simulink library "sm_car_scene_crg_germania_f"  (R2026a)
settings: Solver=VariableStepAuto
undefined symbols (not defined in the file or in its folder): Scene
libraries: Scene_Utilities x3
Description:
  | Scene of Simscape Vehicle Templates Library
  | 
  | Copyright 2018-2024 The MathWorks, Inc.
settings Model: Creator=smiller  LastModifiedBy=andrei

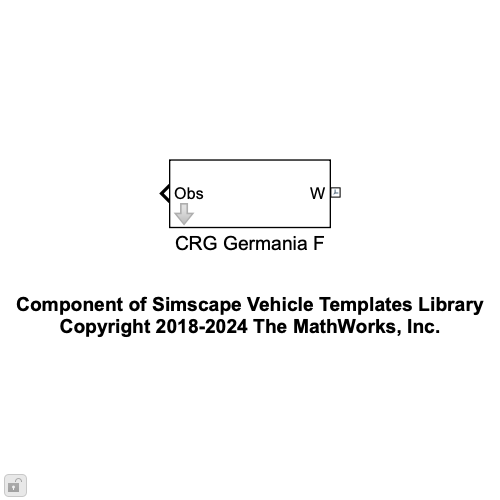
[thumbnail: Simulink's stored preview of the top-level diagram]
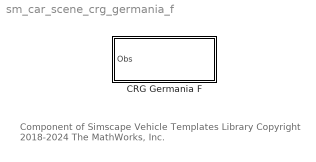
== system sm_car_scene_crg_germania_f ==
  note: Component of Simscape Vehicle Templates Library
      | Copyright 2018-2024 The MathWorks, Inc.
  CRG Germania F : Subsystem  mask{geometry=Scene.CRG_Germania_F.Geometry}
      mask prompts: geometry "Geometry (structure)"

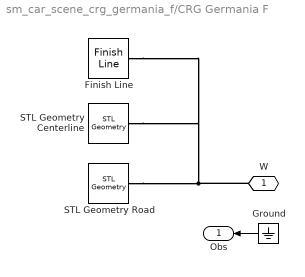
== system sm_car_scene_crg_germania_f/CRG Germania F ==
  Finish Line : Scene_Utilities/Finish Line  post_h=geometry.finish_line.post.height  post_r=geometry.finish_line.post.radius  line_w=geometry.finish_line.post.separation  post_clr=geometry.finish_line.post.clr  post_opc=geometry.finish_line.post.opc  offset_xyz=geometry.finish_line.offset.xyz  offset_yaw=geometry.finish_line.offset.yaw  offset_pitch=geometry.finish_line.offset.pitch  offset_roll=geometry.finish_line.offset.roll
  Ground : Ground
  STL Geometry Centerline : Scene_Utilities/STL Geometry  stl_file=geometry.centerline.filename  stl_units=geometry.centerline.fileunits  stl_clr=geometry.centerline.clr  stl_opc=geometry.centerline.opc  stl_x=geometry.centerline.x  stl_y=geometry.centerline.y  stl_z=geometry.centerline.z  stl_yaw=geometry.centerline.yaw  stl_pitch=geometry.centerline.pitch  stl_roll=geometry.centerline.roll
  STL Geometry Road : Scene_Utilities/STL Geometry  stl_file=geometry.filename  stl_units=geometry.fileunits  stl_clr=geometry.clr  stl_opc=geometry.opc  stl_x=geometry.x  stl_y=geometry.y  stl_z=geometry.z  stl_yaw=geometry.yaw  stl_pitch=geometry.pitch  stl_roll=geometry.roll
  W : PMIOPort  Side=Left
  Obs : Outport  VectorParamsAs1DForOutWhenUnconnected=off
  wires:
  Ground/1 -> Obs/1
  connections:
  STL Geometry Road/RConn1 -- W/RConn1 -- Finish Line/LConn1 -- STL Geometry Centerline/RConn1
